simulink library "lib_LargeBuildingModel"  (R2026a)
settings: Solver=VariableStepAuto
libraries: WallSelector_lib x380, ExternalWall_lib x188, RoomWithAirVolume x140, fl_lib x139, RoomLevelControl_lib x1
(part 1 of 12)
settings Model: Creator=vikrants  LastModifiedBy=vikrants

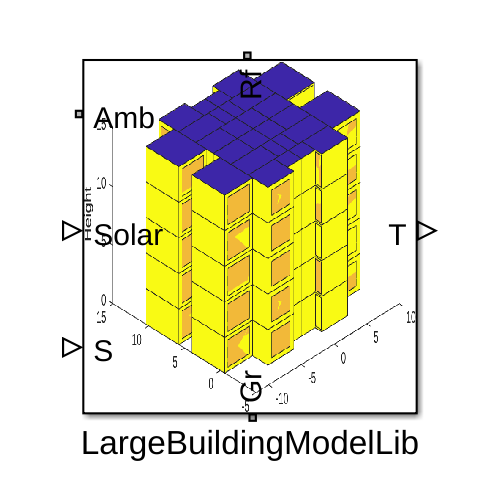
[thumbnail: Simulink's stored preview of the top-level diagram]
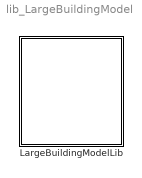
== system lib_LargeBuildingModel ==
  LargeBuildingModelLib : Subsystem
      settings: PortSchema="{\"entries\":[{\"content\":{\"sides\":[{\"content\":{\"connectorIds\":[\"LConn1\",\"LConn2\",\"LConn3\"]},\"type\":\"ConnectorPlacement.EquallySpacedRectSide\",\"uuid\":\"a54174e5-5a1e-4089-b263-99354bf7a073\"},{\"content\":{\"connectorIds\":[\"RConn1\"],\"side\":\"RIGHT\"},\"type\":\"ConnectorPlacement.EquallySpacedRectSide\",\"uuid\":\"c2c2a31f-cd98-4c14-b6c8-dd8555ba1cf6\"},{\"content\":{\"connectorIds\":[\"LConn4\"],\"side\":\"TOP\"},\"type\":\"ConnectorPlacement.EquallySpacedRectSide\",\"uuid\":\"2487b9c5-89a9-4b1a-9c1c-aa8a65c4be64\"},{\"content\":{\"connectorIds\":[\"RConn2\"],\"side\":\"BOTTOM\"},\"type\":\"ConnectorPlacement.EquallySpacedRectSide\",\"uuid\":\"6826558f-5b15-4554-8d35-ce4ee9628e1d\"}]},\"type\":\"ConnectorPlacement.EquallySpacedConnector\",\"uuid\":\"0b65bcf1-6575-4ff3-9247-4f08434b0bb6\"}],\"packageUris\":[\"http://schema.mathworks.com/mf0/Connector/R2020b\"],\"version\":\"1.0\"}"
      mask Display: image('lib_LargeBuildingModel.png')

== system lib_LargeBuildingModel/LargeBuildingModelLib ==
  ConnectLevel0and1 : Subsystem
      settings: PortSchema="{\"entries\":[{\"content\":{\"sides\":[{\"content\":{},\"type\":\"ConnectorPlacement.EquallySpacedRectSide\",\"uuid\":\"bfcbcdaf-7e68-43ba-b21b-739e3d917df2\"},{\"content\":{\"side\":\"RIGHT\"},\"type\":\"ConnectorPlacement.EquallySpacedRectSide\",\"uuid\":\"1db46710-465c-454f-9fe4-f8c04c90b155\"},{\"content\":{\"connectorIds\":[\"LConn1\"],\"side\":\"TOP\"},\"type\":\"ConnectorPlacement.EquallySpacedRectSide\",\"uuid\":\"8ba3322a-28ec-4bcd-a32b-78c0e69bc71f\"},{\"content\":{\"connectorIds\":[\"RConn1\"],\"side\":\"BOTTOM\"},\"type\":\"ConnectorPlacement.EquallySpacedRectSide\",\"uuid\":\"ab838286-00a0-4d85-b927-59d0a4342f32\"}]},\"type\":\"ConnectorPlacement.EquallySpacedConnector\",\"uuid\":\"bc7fd7cc-de66-4685-913a-91b57874b9ec\"}],\"packageUris\":[\"http://schema.mathworks.com/mf0/Connector/R2020b\"],\"version\":\"1.0\"}"
  ConnectLevel1and2 : Subsystem
      settings: PortSchema="{\"entries\":[{\"content\":{\"sides\":[{\"content\":{},\"type\":\"ConnectorPlacement.EquallySpacedRectSide\",\"uuid\":\"bfcbcdaf-7e68-43ba-b21b-739e3d917df2\"},{\"content\":{\"side\":\"RIGHT\"},\"type\":\"ConnectorPlacement.EquallySpacedRectSide\",\"uuid\":\"1db46710-465c-454f-9fe4-f8c04c90b155\"},{\"content\":{\"connectorIds\":[\"LConn1\"],\"side\":\"TOP\"},\"type\":\"ConnectorPlacement.EquallySpacedRectSide\",\"uuid\":\"8ba3322a-28ec-4bcd-a32b-78c0e69bc71f\"},{\"content\":{\"connectorIds\":[\"RConn1\"],\"side\":\"BOTTOM\"},\"type\":\"ConnectorPlacement.EquallySpacedRectSide\",\"uuid\":\"f3ab9cf8-9c6a-48e9-b20b-6fd302e3ecc9\"}]},\"type\":\"ConnectorPlacement.EquallySpacedConnector\",\"uuid\":\"bc7fd7cc-de66-4685-913a-91b57874b9ec\"}],\"packageUris\":[\"http://schema.mathworks.com/mf0/Connector/R2020b\"],\"version\":\"1.0\"}"
  ConnectLevel2and3 : Subsystem
      settings: PortSchema="{\"entries\":[{\"content\":{\"sides\":[{\"content\":{},\"type\":\"ConnectorPlacement.EquallySpacedRectSide\",\"uuid\":\"bfcbcdaf-7e68-43ba-b21b-739e3d917df2\"},{\"content\":{\"side\":\"RIGHT\"},\"type\":\"ConnectorPlacement.EquallySpacedRectSide\",\"uuid\":\"1db46710-465c-454f-9fe4-f8c04c90b155\"},{\"content\":{\"connectorIds\":[\"LConn1\"],\"side\":\"TOP\"},\"type\":\"ConnectorPlacement.EquallySpacedRectSide\",\"uuid\":\"8ba3322a-28ec-4bcd-a32b-78c0e69bc71f\"},{\"content\":{\"connectorIds\":[\"RConn1\"],\"side\":\"BOTTOM\"},\"type\":\"ConnectorPlacement.EquallySpacedRectSide\",\"uuid\":\"f8b3c343-7c17-4a2c-a5df-2d9e42135e3d\"}]},\"type\":\"ConnectorPlacement.EquallySpacedConnector\",\"uuid\":\"bc7fd7cc-de66-4685-913a-91b57874b9ec\"}],\"packageUris\":[\"http://schema.mathworks.com/mf0/Connector/R2020b\"],\"version\":\"1.0\"}"
  ConnectLevel3and4 : Subsystem
      settings: PortSchema="{\"entries\":[{\"content\":{\"sides\":[{\"content\":{},\"type\":\"ConnectorPlacement.EquallySpacedRectSide\",\"uuid\":\"bfcbcdaf-7e68-43ba-b21b-739e3d917df2\"},{\"content\":{\"side\":\"RIGHT\"},\"type\":\"ConnectorPlacement.EquallySpacedRectSide\",\"uuid\":\"1db46710-465c-454f-9fe4-f8c04c90b155\"},{\"content\":{\"connectorIds\":[\"LConn1\"],\"side\":\"TOP\"},\"type\":\"ConnectorPlacement.EquallySpacedRectSide\",\"uuid\":\"8ba3322a-28ec-4bcd-a32b-78c0e69bc71f\"},{\"content\":{\"connectorIds\":[\"RConn1\"],\"side\":\"BOTTOM\"},\"type\":\"ConnectorPlacement.EquallySpacedRectSide\",\"uuid\":\"2c50accd-6f19-4351-b387-00bd4c13865a\"}]},\"type\":\"ConnectorPlacement.EquallySpacedConnector\",\"uuid\":\"bc7fd7cc-de66-4685-913a-91b57874b9ec\"}],\"packageUris\":[\"http://schema.mathworks.com/mf0/Connector/R2020b\"],\"version\":\"1.0\"}"
  Ground : Subsystem
      settings: PortSchema="{\"entries\":[{\"content\":{\"sides\":[{\"content\":{},\"type\":\"ConnectorPlacement.EquallySpacedRectSide\",\"uuid\":\"bfcbcdaf-7e68-43ba-b21b-739e3d917df2\"},{\"content\":{\"side\":\"RIGHT\"},\"type\":\"ConnectorPlacement.EquallySpacedRectSide\",\"uuid\":\"1db46710-465c-454f-9fe4-f8c04c90b155\"},{\"content\":{\"connectorIds\":[\"LConn1\"],\"side\":\"TOP\"},\"type\":\"ConnectorPlacement.EquallySpacedRectSide\",\"uuid\":\"8ba3322a-28ec-4bcd-a32b-78c0e69bc71f\"},{\"content\":{\"connectorIds\":[\"RConn1\"],\"side\":\"BOTTOM\"},\"type\":\"ConnectorPlacement.EquallySpacedRectSide\",\"uuid\":\"e9de58ce-608e-4d22-b435-941c76f225f1\"}]},\"type\":\"ConnectorPlacement.EquallySpacedConnector\",\"uuid\":\"bc7fd7cc-de66-4685-913a-91b57874b9ec\"}],\"packageUris\":[\"http://schema.mathworks.com/mf0/Connector/R2020b\"],\"version\":\"1.0\"}"
  Level0 : Subsystem
      settings: PortSchema="{\"entries\":[{\"content\":{\"sides\":[{\"content\":{\"connectorIds\":[\"LConn1\",\"LConn2\",\"LConn3\"]},\"type\":\"ConnectorPlacement.EquallySpacedRectSide\",\"uuid\":\"f5302b38-994b-4d73-bed8-b19055c1e83a\"},{\"content\":{\"connectorIds\":[\"RConn1\"],\"side\":\"RIGHT\"},\"type\":\"ConnectorPlacement.EquallySpacedRectSide\",\"uuid\":\"faa5d083-f69a-475e-bab7-3d1e14a6968b\"},{\"content\":{\"connectorIds\":[\"LConn4\"],\"side\":\"TOP\"},\"type\":\"ConnectorPlacement.EquallySpacedRectSide\",\"uuid\":\"f79c44c3-41c3-478c-a059-469d9fb7ebbf\"},{\"content\":{\"connectorIds\":[\"RConn2\"],\"side\":\"BOTTOM\"},\"type\":\"ConnectorPlacement.EquallySpacedRectSide\",\"uuid\":\"9239f0d3-0017-4bc4-8897-67227729a1c7\"}]},\"type\":\"ConnectorPlacement.EquallySpacedConnector\",\"uuid\":\"c9eb4cc8-9d3a-4a18-b359-75861972c164\"}],\"packageUris\":[\"http://schema.mathworks.com/mf0/Connector/R2020b\"],\"version\":\"1.0\"}"
  Level1 : Subsystem
      settings: PortSchema="{\"entries\":[{\"content\":{\"sides\":[{\"content\":{\"connectorIds\":[\"LConn1\",\"LConn2\",\"LConn3\"]},\"type\":\"ConnectorPlacement.EquallySpacedRectSide\",\"uuid\":\"f5302b38-994b-4d73-bed8-b19055c1e83a\"},{\"content\":{\"connectorIds\":[\"RConn1\"],\"side\":\"RIGHT\"},\"type\":\"ConnectorPlacement.EquallySpacedRectSide\",\"uuid\":\"faa5d083-f69a-475e-bab7-3d1e14a6968b\"},{\"content\":{\"connectorIds\":[\"LConn4\"],\"side\":\"TOP\"},\"type\":\"ConnectorPlacement.EquallySpacedRectSide\",\"uuid\":\"f79c44c3-41c3-478c-a059-469d9fb7ebbf\"},{\"content\":{\"connectorIds\":[\"RConn2\"],\"side\":\"BOTTOM\"},\"type\":\"ConnectorPlacement.EquallySpacedRectSide\",\"uuid\":\"a0801537-0af0-4bd5-9c9a-f5991b45aca8\"}]},\"type\":\"ConnectorPlacement.EquallySpacedConnector\",\"uuid\":\"c9eb4cc8-9d3a-4a18-b359-75861972c164\"}],\"packageUris\":[\"http://schema.mathworks.com/mf0/Connector/R2020b\"],\"version\":\"1.0\"}"
  Level2 : Subsystem
      settings: PortSchema="{\"entries\":[{\"content\":{\"sides\":[{\"content\":{\"connectorIds\":[\"LConn1\",\"LConn2\",\"LConn3\"]},\"type\":\"ConnectorPlacement.EquallySpacedRectSide\",\"uuid\":\"f5302b38-994b-4d73-bed8-b19055c1e83a\"},{\"content\":{\"connectorIds\":[\"RConn1\"],\"side\":\"RIGHT\"},\"type\":\"ConnectorPlacement.EquallySpacedRectSide\",\"uuid\":\"faa5d083-f69a-475e-bab7-3d1e14a6968b\"},{\"content\":{\"connectorIds\":[\"LConn4\"],\"side\":\"TOP\"},\"type\":\"ConnectorPlacement.EquallySpacedRectSide\",\"uuid\":\"f79c44c3-41c3-478c-a059-469d9fb7ebbf\"},{\"content\":{\"connectorIds\":[\"RConn2\"],\"side\":\"BOTTOM\"},\"type\":\"ConnectorPlacement.EquallySpacedRectSide\",\"uuid\":\"bd08f839-c923-45c8-997c-e7bb9423b19d\"}]},\"type\":\"ConnectorPlacement.EquallySpacedConnector\",\"uuid\":\"c9eb4cc8-9d3a-4a18-b359-75861972c164\"}],\"packageUris\":[\"http://schema.mathworks.com/mf0/Connector/R2020b\"],\"version\":\"1.0\"}"
  Level3 : Subsystem
      settings: PortSchema="{\"entries\":[{\"content\":{\"sides\":[{\"content\":{\"connectorIds\":[\"LConn1\",\"LConn2\",\"LConn3\"]},\"type\":\"ConnectorPlacement.EquallySpacedRectSide\",\"uuid\":\"f5302b38-994b-4d73-bed8-b19055c1e83a\"},{\"content\":{\"connectorIds\":[\"RConn1\"],\"side\":\"RIGHT\"},\"type\":\"ConnectorPlacement.EquallySpacedRectSide\",\"uuid\":\"faa5d083-f69a-475e-bab7-3d1e14a6968b\"},{\"content\":{\"connectorIds\":[\"LConn4\"],\"side\":\"TOP\"},\"type\":\"ConnectorPlacement.EquallySpacedRectSide\",\"uuid\":\"f79c44c3-41c3-478c-a059-469d9fb7ebbf\"},{\"content\":{\"connectorIds\":[\"RConn2\"],\"side\":\"BOTTOM\"},\"type\":\"ConnectorPlacement.EquallySpacedRectSide\",\"uuid\":\"6ad92d71-3c8c-43ae-8be8-bbeacb5a4479\"}]},\"type\":\"ConnectorPlacement.EquallySpacedConnector\",\"uuid\":\"c9eb4cc8-9d3a-4a18-b359-75861972c164\"}],\"packageUris\":[\"http://schema.mathworks.com/mf0/Connector/R2020b\"],\"version\":\"1.0\"}"
  Level4 : Subsystem
      settings: PortSchema="{\"entries\":[{\"content\":{\"sides\":[{\"content\":{\"connectorIds\":[\"LConn1\",\"LConn2\",\"LConn3\"]},\"type\":\"ConnectorPlacement.EquallySpacedRectSide\",\"uuid\":\"f5302b38-994b-4d73-bed8-b19055c1e83a\"},{\"content\":{\"connectorIds\":[\"RConn1\"],\"side\":\"RIGHT\"},\"type\":\"ConnectorPlacement.EquallySpacedRectSide\",\"uuid\":\"faa5d083-f69a-475e-bab7-3d1e14a6968b\"},{\"content\":{\"connectorIds\":[\"LConn4\"],\"side\":\"TOP\"},\"type\":\"ConnectorPlacement.EquallySpacedRectSide\",\"uuid\":\"f79c44c3-41c3-478c-a059-469d9fb7ebbf\"},{\"content\":{\"connectorIds\":[\"RConn2\"],\"side\":\"BOTTOM\"},\"type\":\"ConnectorPlacement.EquallySpacedRectSide\",\"uuid\":\"444ccc88-7c7b-4932-a02b-9df645918112\"}]},\"type\":\"ConnectorPlacement.EquallySpacedConnector\",\"uuid\":\"c9eb4cc8-9d3a-4a18-b359-75861972c164\"}],\"packageUris\":[\"http://schema.mathworks.com/mf0/Connector/R2020b\"],\"version\":\"1.0\"}"
  Roof : Subsystem
      settings: PortSchema="{\"entries\":[{\"content\":{\"sides\":[{\"content\":{\"connectorIds\":[\"LConn1\"]},\"type\":\"ConnectorPlacement.EquallySpacedRectSide\",\"uuid\":\"330a1f4c-788b-45d3-8144-461e13e4bc2b\"},{\"content\":{\"side\":\"RIGHT\"},\"type\":\"ConnectorPlacement.EquallySpacedRectSide\",\"uuid\":\"2ff68f0e-d161-486d-a47e-10633b293a9f\"},{\"content\":{\"connectorIds\":[\"LConn2\"],\"side\":\"TOP\"},\"type\":\"ConnectorPlacement.EquallySpacedRectSide\",\"uuid\":\"a18254b5-007e-4575-8004-ea2058ac2122\"},{\"content\":{\"connectorIds\":[\"RConn1\"],\"side\":\"BOTTOM\"},\"type\":\"ConnectorPlacement.EquallySpacedRectSide\",\"uuid\":\"9d9d06c4-f9b4-44db-a6ff-ed6ffbc85269\"}]},\"type\":\"ConnectorPlacement.EquallySpacedConnector\",\"uuid\":\"c0f19b20-ad71-4ed9-8cf3-6c486454730f\"}],\"packageUris\":[\"http://schema.mathworks.com/mf0/Connector/R2020b\"],\"version\":\"1.0\"}"
  Sv : RoomLevelControl_lib/Room Level Control  portOption=roomControlOption.heat  roomMapping=[1 1 1 1;1 1 2 2;1 1 3 3;1 1 4 4;1 1 5 5;1 1 6 6;1 1 7 7;1 2 1 8;1 2 2 9;1 2 3 10;1 2 4 11;1 2 5 12;1 2 6 13;1 2 7 14;1 3 1 15;1 3 2 16;1 3 3 17;1 3 4 18;1 3 5 19;1 3 6 20;1 3 7 21;1 4 1 22;1 4 2 23;1 4 3 24;1 4 4 25;1 4 5 26;1 4 6 27;1 4 7 28;2 5 1 29;2 5 2 30;2 5 3 31;2 5 4 32;2 5 5 33;2 5 6 34;2 5 7 35;2 6 1 36;2 6 2 37;2 6 3 38;2 6 4 39;2 6 5 40;2 6 6 41;2 6 7 42;2 7 1 43;2 7 2 44;2 7 3 45;2 7 4 46;2 7 5 47;2 7 6 48;2 7 7 49;2 8 1 50;2 8 2 51;2 8 3 52;2 8 4 53;2 8 5 54;2 8 6 55;2 8 7 56;3 9 1 57;3 9 2 58;3 9 3 59;3 9 4 60;3 9 5 61;3 9 6 62;3 9 7 63;3 10 1 64;3 10 2 65;3 10 3 66;3 10 4 67;3 10 5 68;3 10 6 69;3 10 7 70;3 11 1 71;3 11 2 72;3 11 3 73;3 11 4 74;3 11 5 75;3 11 6 76;3 11 7 77;3 12 1 78;3 12 2 79;3 12 3 80;3 12 4 81;3 12 5 82;3 12 6 83;3 12 7 84;4 13 1 85;4 13 2 86;4 13 3 87;4 13 4 88;4 13 5 89;4 13 6 90;4 13 7 91;4 14 1 92;4 14 2 93;4 14 3 94;4 14 4 95;4 14 5 96;4 14 6 97;4 14 7 98;4 15 1 99;4 15 2 100;4 15 3 101;4 15 4 102;4 15 5 103;4 15 6 104;4 15 7 105;4 16 1 106;4 16 2 107;4 16 3 108;4 16 4 109;4 16 5 110;4 16 6 111;4 16 7 112;5 17 1 113;5 17 2 114;5 17 3 115;5 17 4 116;5 17 5 117;5 17 6 118;5 17 7 119;5 18 1 120;5 18 2 121;5 18 3 122;5 18 4 123;5 18 5 124;5 18 6 125;5 18 7 126;5 19 1 127;5 19 2 128;5 19 3 129;5 19 4 130;5 19 5 131;5 19 6 132;5 19 7 133;5 20 1 134;5 20 2 135;5 20 3 136;5 20 4 137;5 20 5 138;5 20 6 139;5 20 7 140]
  roomT : Subsystem
  Amb : PMIOPort  Side=Left
  Solar : PMIOPort  Port=2  Side=Left
  S : PMIOPort  Port=3  Side=Left
  Rf : PMIOPort  Port=4  Side=Left
  T : PMIOPort  Port=5  Side=Right
  Gr : PMIOPort  Port=6  Side=Right
  connections:
  Level0/RConn2 -- Ground/LConn1
  Level1/RConn2 -- ConnectLevel0and1/LConn1
  Level0/LConn4 -- ConnectLevel0and1/RConn1
  Level2/RConn2 -- ConnectLevel1and2/LConn1
  Level1/LConn4 -- ConnectLevel1and2/RConn1
  Level3/RConn2 -- ConnectLevel2and3/LConn1
  Level2/LConn4 -- ConnectLevel2and3/RConn1
  Level4/RConn2 -- ConnectLevel3and4/LConn1
  Level3/LConn4 -- ConnectLevel3and4/RConn1
  Level4/LConn4 -- Roof/RConn1
  Sv/LConn1 -- S/RConn1
  Roof/LConn2 -- Rf/RConn1
  Ground/RConn1 -- Gr/RConn1
  Roof/LConn1 -- Level0/LConn2 -- Level1/LConn2 -- Level2/LConn2 -- Level3/LConn2 -- Solar/RConn1 -- Level4/LConn2
  Level0/LConn1 -- Level1/LConn1 -- Level2/LConn1 -- Level3/LConn1 -- Amb/RConn1 -- Level4/LConn1
  Level0/LConn3 -- Level1/LConn3 -- Level2/LConn3 -- Level3/LConn3 -- Sv/RConn1 -- Level4/LConn3
  roomT/LConn1 -- Level0/RConn1
  roomT/LConn2 -- Level1/RConn1
  roomT/LConn3 -- Level2/RConn1
  roomT/LConn4 -- Level3/RConn1
  roomT/LConn5 -- Level4/RConn1
  roomT/RConn1 -- T/RConn1

== system lib_LargeBuildingModel/LargeBuildingModelLib/ConnectLevel0and1 ==
  note: Floor_A1R1(LivingRoom_A)
  note: Floor_A1R2(Bedroom_A)
  note: Floor_A1R3(Kitchen_A)
  note: Floor_A1R4(Bathroom_A)
  note: Floor_A1R5(FireExit_A)
  note: Floor_A1R6(Lobby1_A)
  note: Floor_A1R7(Lobby2_A)
  note: Floor_A2R1(LivingRoom_B)
  note: Floor_A2R2(Bedroom_B)
  note: Floor_A2R3(Kitchen_B)
  note: Floor_A2R4(Bathroom_B)
  note: Floor_A2R5(FireExit_B)
  note: Floor_A2R6(Lobby1_B)
  note: Floor_A2R7(Lobby2_B)
  note: Floor_A3R1(LivingRoom_C)
  note: Floor_A3R2(Bedroom_C)
  note: Floor_A3R3(Kitchen_C)
  note: Floor_A3R4(Bathroom_C)
  note: Floor_A3R5(FireExit_C)
  note: Floor_A3R6(Lobby1_C)
  note: Floor_A3R7(Lobby2_C)
  note: Floor_A4R1(LivingRoom_D)
  note: Floor_A4R2(Bedroom_D)
  note: Floor_A4R3(Kitchen_D)
  note: Floor_A4R4(Bathroom_D)
  note: Floor_A4R5(FireExit_D)
  note: Floor_A4R6(Lobby1_D)
  note: Floor_A4R7(Lobby2_D)
  ArrayBottom : SimscapeArrayConnection  Domain=foundation.thermal.thermal  ConcatenateDimension=1  NumScalarElements=28
  ArrayTop : SimscapeArrayConnection  Domain=foundation.thermal.thermal  ConcatenateDimension=1  NumScalarElements=28
  Floor_A1R1(LivingRoom_A)Blk : WallSelector_lib/Wall Selector  optWall=wallModelOption.wallOnly  wallLength=2.4384 % Parameterized on : 13-Jun-2026 10:47:15 m  wallHeight=4.572 % Parameterized on : 13-Jun-2026 10:47:15 m  wallThickness=0.03 % Parameterized on : 13-Jun-2026 10:47:15 m  wallMaterialDen=1400 % Parameterized on : 13-Jun-2026 10:47:28 kg/m^3  wallMaterialCp=1000 % Parameterized on : 13-Jun-2026 10:47:28 J/(K*kg)  wallAbsorptivity=0.5  wallThermalK=0.7 % Parameterized on : 13-Jun-2026 10:47:28 W/(K*m)  winLength=1 m  winHeight=0.5 m  winThickness=0.007 m  winMaterialDen=2500 kg/m^3  winMaterialCp=787 J/(K*kg)  winAbsorptivity=0.35  winThermalK=1 W/(K*m)  winTransmissivity=0.45  ventLength=0.1 m  ventHeight=0.1 m  extToWallHTC=30 % Parameterized on : 13-Jun-2026 10:47:28 W/(K*m^2)  intToRoomHTC=30 % Parameterized on : 13-Jun-2026 10:47:28 W/(K*m^2)  iniT=300 % Parameterized on : 13-Jun-2026 10:47:28 K
  Floor_A1R2(Bedroom_A)Blk : WallSelector_lib/Wall Selector  optWall=wallModelOption.wallOnly  wallLength=4.2672 % Parameterized on : 13-Jun-2026 10:47:15 m  wallHeight=4.572 % Parameterized on : 13-Jun-2026 10:47:15 m  wallThickness=0.03 % Parameterized on : 13-Jun-2026 10:47:15 m  wallMaterialDen=1400 % Parameterized on : 13-Jun-2026 10:47:28 kg/m^3  wallMaterialCp=1000 % Parameterized on : 13-Jun-2026 10:47:28 J/(K*kg)  wallAbsorptivity=0.5  wallThermalK=0.7 % Parameterized on : 13-Jun-2026 10:47:28 W/(K*m)  winLength=1 m  winHeight=0.5 m  winThickness=0.007 m  winMaterialDen=2500 kg/m^3  winMaterialCp=787 J/(K*kg)  winAbsorptivity=0.35  winThermalK=1 W/(K*m)  winTransmissivity=0.45  ventLength=0.1 m  ventHeight=0.1 m  extToWallHTC=30 % Parameterized on : 13-Jun-2026 10:47:28 W/(K*m^2)  intToRoomHTC=30 % Parameterized on : 13-Jun-2026 10:47:28 W/(K*m^2)  iniT=300 % Parameterized on : 13-Jun-2026 10:47:28 K
  Floor_A1R3(Kitchen_A)Blk : WallSelector_lib/Wall Selector  optWall=wallModelOption.wallOnly  wallLength=2.7432 % Parameterized on : 13-Jun-2026 10:47:15 m  wallHeight=3.9624 % Parameterized on : 13-Jun-2026 10:47:15 m  wallThickness=0.03 % Parameterized on : 13-Jun-2026 10:47:15 m  wallMaterialDen=1400 % Parameterized on : 13-Jun-2026 10:47:28 kg/m^3  wallMaterialCp=1000 % Parameterized on : 13-Jun-2026 10:47:28 J/(K*kg)  wallAbsorptivity=0.5  wallThermalK=0.7 % Parameterized on : 13-Jun-2026 10:47:28 W/(K*m)  winLength=1 m  winHeight=0.5 m  winThickness=0.007 m  winMaterialDen=2500 kg/m^3  winMaterialCp=787 J/(K*kg)  winAbsorptivity=0.35  winThermalK=1 W/(K*m)  winTransmissivity=0.45  ventLength=0.1 m  ventHeight=0.1 m  extToWallHTC=30 % Parameterized on : 13-Jun-2026 10:47:28 W/(K*m^2)  intToRoomHTC=30 % Parameterized on : 13-Jun-2026 10:47:28 W/(K*m^2)  iniT=300 % Parameterized on : 13-Jun-2026 10:47:28 K
  Floor_A1R4(Bathroom_A)Blk : WallSelector_lib/Wall Selector  optWall=wallModelOption.wallOnly  wallLength=2.4384 % Parameterized on : 13-Jun-2026 10:47:15 m  wallHeight=3.6576 % Parameterized on : 13-Jun-2026 10:47:15 m  wallThickness=0.03 % Parameterized on : 13-Jun-2026 10:47:15 m  wallMaterialDen=1400 % Parameterized on : 13-Jun-2026 10:47:28 kg/m^3  wallMaterialCp=1000 % Parameterized on : 13-Jun-2026 10:47:28 J/(K*kg)  wallAbsorptivity=0.5  wallThermalK=0.7 % Parameterized on : 13-Jun-2026 10:47:28 W/(K*m)  winLength=1 m  winHeight=0.5 m  winThickness=0.007 m  winMaterialDen=2500 kg/m^3  winMaterialCp=787 J/(K*kg)  winAbsorptivity=0.35  winThermalK=1 W/(K*m)  winTransmissivity=0.45  ventLength=0.1 m  ventHeight=0.1 m  extToWallHTC=30 % Parameterized on : 13-Jun-2026 10:47:28 W/(K*m^2)  intToRoomHTC=30 % Parameterized on : 13-Jun-2026 10:47:28 W/(K*m^2)  iniT=300 % Parameterized on : 13-Jun-2026 10:47:28 K
  Floor_A1R5(FireExit_A)Blk : WallSelector_lib/Wall Selector  optWall=wallModelOption.wallOnly  wallLength=1.8288 % Parameterized on : 13-Jun-2026 10:47:15 m  wallHeight=2.1336 % Parameterized on : 13-Jun-2026 10:47:15 m  wallThickness=0.03 % Parameterized on : 13-Jun-2026 10:47:15 m  wallMaterialDen=1400 % Parameterized on : 13-Jun-2026 10:47:28 kg/m^3  wallMaterialCp=1000 % Parameterized on : 13-Jun-2026 10:47:28 J/(K*kg)  wallAbsorptivity=0.5  wallThermalK=0.7 % Parameterized on : 13-Jun-2026 10:47:28 W/(K*m)  winLength=1 m  winHeight=0.5 m  winThickness=0.007 m  winMaterialDen=2500 kg/m^3  winMaterialCp=787 J/(K*kg)  winAbsorptivity=0.35  winThermalK=1 W/(K*m)  winTransmissivity=0.45  ventLength=0.1 m  ventHeight=0.1 m  extToWallHTC=30 % Parameterized on : 13-Jun-2026 10:47:28 W/(K*m^2)  intToRoomHTC=30 % Parameterized on : 13-Jun-2026 10:47:28 W/(K*m^2)  iniT=300 % Parameterized on : 13-Jun-2026 10:47:28 K
  Floor_A1R6(Lobby1_A)Blk : WallSelector_lib/Wall Selector  optWall=wallModelOption.wallOnly  wallLength=2.4384 % Parameterized on : 13-Jun-2026 10:47:15 m  wallHeight=2.4384 % Parameterized on : 13-Jun-2026 10:47:15 m  wallThickness=0.03 % Parameterized on : 13-Jun-2026 10:47:15 m  wallMaterialDen=1400 % Parameterized on : 13-Jun-2026 10:47:28 kg/m^3  wallMaterialCp=1000 % Parameterized on : 13-Jun-2026 10:47:28 J/(K*kg)  wallAbsorptivity=0.5  wallThermalK=0.7 % Parameterized on : 13-Jun-2026 10:47:28 W/(K*m)  winLength=1 m  winHeight=0.5 m  winThickness=0.007 m  winMaterialDen=2500 kg/m^3  winMaterialCp=787 J/(K*kg)  winAbsorptivity=0.35  winThermalK=1 W/(K*m)  winTransmissivity=0.45  ventLength=0.1 m  ventHeight=0.1 m  extToWallHTC=30 % Parameterized on : 13-Jun-2026 10:47:28 W/(K*m^2)  intToRoomHTC=30 % Parameterized on : 13-Jun-2026 10:47:28 W/(K*m^2)  iniT=300 % Parameterized on : 13-Jun-2026 10:47:28 K
  Floor_A1R7(Lobby2_A)Blk : WallSelector_lib/Wall Selector  optWall=wallModelOption.wallOnly  wallLength=2.4384 % Parameterized on : 13-Jun-2026 10:47:15 m  wallHeight=1.524 % Parameterized on : 13-Jun-2026 10:47:15 m  wallThickness=0.03 % Parameterized on : 13-Jun-2026 10:47:15 m  wallMaterialDen=1400 % Parameterized on : 13-Jun-2026 10:47:28 kg/m^3  wallMaterialCp=1000 % Parameterized on : 13-Jun-2026 10:47:28 J/(K*kg)  wallAbsorptivity=0.5  wallThermalK=0.7 % Parameterized on : 13-Jun-2026 10:47:28 W/(K*m)  winLength=1 m  winHeight=0.5 m  winThickness=0.007 m  winMaterialDen=2500 kg/m^3  winMaterialCp=787 J/(K*kg)  winAbsorptivity=0.35  winThermalK=1 W/(K*m)  winTransmissivity=0.45  ventLength=0.1 m  ventHeight=0.1 m  extToWallHTC=30 % Parameterized on : 13-Jun-2026 10:47:28 W/(K*m^2)  intToRoomHTC=30 % Parameterized on : 13-Jun-2026 10:47:28 W/(K*m^2)  iniT=300 % Parameterized on : 13-Jun-2026 10:47:28 K
  Floor_A2R1(LivingRoom_B)Blk : WallSelector_lib/Wall Selector  optWall=wallModelOption.wallOnly  wallLength=2.4384 % Parameterized on : 13-Jun-2026 10:47:15 m  wallHeight=4.572 % Parameterized on : 13-Jun-2026 10:47:15 m  wallThickness=0.03 % Parameterized on : 13-Jun-2026 10:47:15 m  wallMaterialDen=1400 % Parameterized on : 13-Jun-2026 10:47:29 kg/m^3  wallMaterialCp=1000 % Parameterized on : 13-Jun-2026 10:47:29 J/(K*kg)  wallAbsorptivity=0.5  wallThermalK=0.7 % Parameterized on : 13-Jun-2026 10:47:29 W/(K*m)  winLength=1 m  winHeight=0.5 m  winThickness=0.007 m  winMaterialDen=2500 kg/m^3  winMaterialCp=787 J/(K*kg)  winAbsorptivity=0.35  winThermalK=1 W/(K*m)  winTransmissivity=0.45  ventLength=0.1 m  ventHeight=0.1 m  extToWallHTC=30 % Parameterized on : 13-Jun-2026 10:47:29 W/(K*m^2)  intToRoomHTC=30 % Parameterized on : 13-Jun-2026 10:47:29 W/(K*m^2)  iniT=300 % Parameterized on : 13-Jun-2026 10:47:29 K
  Floor_A2R2(Bedroom_B)Blk : WallSelector_lib/Wall Selector  optWall=wallModelOption.wallOnly  wallLength=4.2672 % Parameterized on : 13-Jun-2026 10:47:15 m  wallHeight=4.572 % Parameterized on : 13-Jun-2026 10:47:15 m  wallThickness=0.03 % Parameterized on : 13-Jun-2026 10:47:15 m  wallMaterialDen=1400 % Parameterized on : 13-Jun-2026 10:47:29 kg/m^3  wallMaterialCp=1000 % Parameterized on : 13-Jun-2026 10:47:29 J/(K*kg)  wallAbsorptivity=0.5  wallThermalK=0.7 % Parameterized on : 13-Jun-2026 10:47:29 W/(K*m)  winLength=1 m  winHeight=0.5 m  winThickness=0.007 m  winMaterialDen=2500 kg/m^3  winMaterialCp=787 J/(K*kg)  winAbsorptivity=0.35  winThermalK=1 W/(K*m)  winTransmissivity=0.45  ventLength=0.1 m  ventHeight=0.1 m  extToWallHTC=30 % Parameterized on : 13-Jun-2026 10:47:29 W/(K*m^2)  intToRoomHTC=30 % Parameterized on : 13-Jun-2026 10:47:29 W/(K*m^2)  iniT=300 % Parameterized on : 13-Jun-2026 10:47:29 K
  Floor_A2R3(Kitchen_B)Blk : WallSelector_lib/Wall Selector  optWall=wallModelOption.wallOnly  wallLength=2.7432 % Parameterized on : 13-Jun-2026 10:47:15 m  wallHeight=3.9624 % Parameterized on : 13-Jun-2026 10:47:15 m  wallThickness=0.03 % Parameterized on : 13-Jun-2026 10:47:15 m  wallMaterialDen=1400 % Parameterized on : 13-Jun-2026 10:47:29 kg/m^3  wallMaterialCp=1000 % Parameterized on : 13-Jun-2026 10:47:29 J/(K*kg)  wallAbsorptivity=0.5  wallThermalK=0.7 % Parameterized on : 13-Jun-2026 10:47:29 W/(K*m)  winLength=1 m  winHeight=0.5 m  winThickness=0.007 m  winMaterialDen=2500 kg/m^3  winMaterialCp=787 J/(K*kg)  winAbsorptivity=0.35  winThermalK=1 W/(K*m)  winTransmissivity=0.45  ventLength=0.1 m  ventHeight=0.1 m  extToWallHTC=30 % Parameterized on : 13-Jun-2026 10:47:29 W/(K*m^2)  intToRoomHTC=30 % Parameterized on : 13-Jun-2026 10:47:29 W/(K*m^2)  iniT=300 % Parameterized on : 13-Jun-2026 10:47:29 K
  Floor_A2R4(Bathroom_B)Blk : WallSelector_lib/Wall Selector  optWall=wallModelOption.wallOnly  wallLength=2.4384 % Parameterized on : 13-Jun-2026 10:47:15 m  wallHeight=3.6576 % Parameterized on : 13-Jun-2026 10:47:15 m  wallThickness=0.03 % Parameterized on : 13-Jun-2026 10:47:15 m  wallMaterialDen=1400 % Parameterized on : 13-Jun-2026 10:47:29 kg/m^3  wallMaterialCp=1000 % Parameterized on : 13-Jun-2026 10:47:29 J/(K*kg)  wallAbsorptivity=0.5  wallThermalK=0.7 % Parameterized on : 13-Jun-2026 10:47:29 W/(K*m)  winLength=1 m  winHeight=0.5 m  winThickness=0.007 m  winMaterialDen=2500 kg/m^3  winMaterialCp=787 J/(K*kg)  winAbsorptivity=0.35  winThermalK=1 W/(K*m)  winTransmissivity=0.45  ventLength=0.1 m  ventHeight=0.1 m  extToWallHTC=30 % Parameterized on : 13-Jun-2026 10:47:29 W/(K*m^2)  intToRoomHTC=30 % Parameterized on : 13-Jun-2026 10:47:29 W/(K*m^2)  iniT=300 % Parameterized on : 13-Jun-2026 10:47:29 K
  Floor_A2R5(FireExit_B)Blk : WallSelector_lib/Wall Selector  optWall=wallModelOption.wallOnly  wallLength=1.8288 % Parameterized on : 13-Jun-2026 10:47:15 m  wallHeight=2.1336 % Parameterized on : 13-Jun-2026 10:47:15 m  wallThickness=0.03 % Parameterized on : 13-Jun-2026 10:47:15 m  wallMaterialDen=1400 % Parameterized on : 13-Jun-2026 10:47:29 kg/m^3  wallMaterialCp=1000 % Parameterized on : 13-Jun-2026 10:47:29 J/(K*kg)  wallAbsorptivity=0.5  wallThermalK=0.7 % Parameterized on : 13-Jun-2026 10:47:29 W/(K*m)  winLength=1 m  winHeight=0.5 m  winThickness=0.007 m  winMaterialDen=2500 kg/m^3  winMaterialCp=787 J/(K*kg)  winAbsorptivity=0.35  winThermalK=1 W/(K*m)  winTransmissivity=0.45  ventLength=0.1 m  ventHeight=0.1 m  extToWallHTC=30 % Parameterized on : 13-Jun-2026 10:47:29 W/(K*m^2)  intToRoomHTC=30 % Parameterized on : 13-Jun-2026 10:47:29 W/(K*m^2)  iniT=300 % Parameterized on : 13-Jun-2026 10:47:29 K
  Floor_A2R6(Lobby1_B)Blk : WallSelector_lib/Wall Selector  optWall=wallModelOption.wallOnly  wallLength=2.4384 % Parameterized on : 13-Jun-2026 10:47:15 m  wallHeight=2.4384 % Parameterized on : 13-Jun-2026 10:47:15 m  wallThickness=0.03 % Parameterized on : 13-Jun-2026 10:47:15 m  wallMaterialDen=1400 % Parameterized on : 13-Jun-2026 10:47:29 kg/m^3  wallMaterialCp=1000 % Parameterized on : 13-Jun-2026 10:47:29 J/(K*kg)  wallAbsorptivity=0.5  wallThermalK=0.7 % Parameterized on : 13-Jun-2026 10:47:29 W/(K*m)  winLength=1 m  winHeight=0.5 m  winThickness=0.007 m  winMaterialDen=2500 kg/m^3  winMaterialCp=787 J/(K*kg)  winAbsorptivity=0.35  winThermalK=1 W/(K*m)  winTransmissivity=0.45  ventLength=0.1 m  ventHeight=0.1 m  extToWallHTC=30 % Parameterized on : 13-Jun-2026 10:47:29 W/(K*m^2)  intToRoomHTC=30 % Parameterized on : 13-Jun-2026 10:47:29 W/(K*m^2)  iniT=300 % Parameterized on : 13-Jun-2026 10:47:29 K
  Floor_A2R7(Lobby2_B)Blk : WallSelector_lib/Wall Selector  optWall=wallModelOption.wallOnly  wallLength=2.4384 % Parameterized on : 13-Jun-2026 10:47:15 m  wallHeight=1.524 % Parameterized on : 13-Jun-2026 10:47:15 m  wallThickness=0.03 % Parameterized on : 13-Jun-2026 10:47:15 m  wallMaterialDen=1400 % Parameterized on : 13-Jun-2026 10:47:29 kg/m^3  wallMaterialCp=1000 % Parameterized on : 13-Jun-2026 10:47:29 J/(K*kg)  wallAbsorptivity=0.5  wallThermalK=0.7 % Parameterized on : 13-Jun-2026 10:47:29 W/(K*m)  winLength=1 m  winHeight=0.5 m  winThickness=0.007 m  winMaterialDen=2500 kg/m^3  winMaterialCp=787 J/(K*kg)  winAbsorptivity=0.35  winThermalK=1 W/(K*m)  winTransmissivity=0.45  ventLength=0.1 m  ventHeight=0.1 m  extToWallHTC=30 % Parameterized on : 13-Jun-2026 10:47:29 W/(K*m^2)  intToRoomHTC=30 % Parameterized on : 13-Jun-2026 10:47:29 W/(K*m^2)  iniT=300 % Parameterized on : 13-Jun-2026 10:47:29 K
  Floor_A3R1(LivingRoom_C)Blk : WallSelector_lib/Wall Selector  optWall=wallModelOption.wallOnly  wallLength=2.4384 % Parameterized on : 13-Jun-2026 10:47:15 m  wallHeight=4.572 % Parameterized on : 13-Jun-2026 10:47:15 m  wallThickness=0.03 % Parameterized on : 13-Jun-2026 10:47:15 m  wallMaterialDen=1400 % Parameterized on : 13-Jun-2026 10:47:29 kg/m^3  wallMaterialCp=1000 % Parameterized on : 13-Jun-2026 10:47:29 J/(K*kg)  wallAbsorptivity=0.5  wallThermalK=0.7 % Parameterized on : 13-Jun-2026 10:47:29 W/(K*m)  winLength=1 m  winHeight=0.5 m  winThickness=0.007 m  winMaterialDen=2500 kg/m^3  winMaterialCp=787 J/(K*kg)  winAbsorptivity=0.35  winThermalK=1 W/(K*m)  winTransmissivity=0.45  ventLength=0.1 m  ventHeight=0.1 m  extToWallHTC=30 % Parameterized on : 13-Jun-2026 10:47:29 W/(K*m^2)  intToRoomHTC=30 % Parameterized on : 13-Jun-2026 10:47:29 W/(K*m^2)  iniT=300 % Parameterized on : 13-Jun-2026 10:47:29 K
  Floor_A3R2(Bedroom_C)Blk : WallSelector_lib/Wall Selector  optWall=wallModelOption.wallOnly  wallLength=4.2672 % Parameterized on : 13-Jun-2026 10:47:15 m  wallHeight=4.572 % Parameterized on : 13-Jun-2026 10:47:15 m  wallThickness=0.03 % Parameterized on : 13-Jun-2026 10:47:15 m  wallMaterialDen=1400 % Parameterized on : 13-Jun-2026 10:47:29 kg/m^3  wallMaterialCp=1000 % Parameterized on : 13-Jun-2026 10:47:29 J/(K*kg)  wallAbsorptivity=0.5  wallThermalK=0.7 % Parameterized on : 13-Jun-2026 10:47:29 W/(K*m)  winLength=1 m  winHeight=0.5 m  winThickness=0.007 m  winMaterialDen=2500 kg/m^3  winMaterialCp=787 J/(K*kg)  winAbsorptivity=0.35  winThermalK=1 W/(K*m)  winTransmissivity=0.45  ventLength=0.1 m  ventHeight=0.1 m  extToWallHTC=30 % Parameterized on : 13-Jun-2026 10:47:29 W/(K*m^2)  intToRoomHTC=30 % Parameterized on : 13-Jun-2026 10:47:29 W/(K*m^2)  iniT=300 % Parameterized on : 13-Jun-2026 10:47:29 K
  Floor_A3R3(Kitchen_C)Blk : WallSelector_lib/Wall Selector  optWall=wallModelOption.wallOnly  wallLength=2.7432 % Parameterized on : 13-Jun-2026 10:47:15 m  wallHeight=3.9624 % Parameterized on : 13-Jun-2026 10:47:15 m  wallThickness=0.03 % Parameterized on : 13-Jun-2026 10:47:15 m  wallMaterialDen=1400 % Parameterized on : 13-Jun-2026 10:47:29 kg/m^3  wallMaterialCp=1000 % Parameterized on : 13-Jun-2026 10:47:29 J/(K*kg)  wallAbsorptivity=0.5  wallThermalK=0.7 % Parameterized on : 13-Jun-2026 10:47:29 W/(K*m)  winLength=1 m  winHeight=0.5 m  winThickness=0.007 m  winMaterialDen=2500 kg/m^3  winMaterialCp=787 J/(K*kg)  winAbsorptivity=0.35  winThermalK=1 W/(K*m)  winTransmissivity=0.45  ventLength=0.1 m  ventHeight=0.1 m  extToWallHTC=30 % Parameterized on : 13-Jun-2026 10:47:29 W/(K*m^2)  intToRoomHTC=30 % Parameterized on : 13-Jun-2026 10:47:29 W/(K*m^2)  iniT=300 % Parameterized on : 13-Jun-2026 10:47:29 K
  Floor_A3R4(Bathroom_C)Blk : WallSelector_lib/Wall Selector  optWall=wallModelOption.wallOnly  wallLength=2.4384 % Parameterized on : 13-Jun-2026 10:47:15 m  wallHeight=3.6576 % Parameterized on : 13-Jun-2026 10:47:15 m  wallThickness=0.03 % Parameterized on : 13-Jun-2026 10:47:15 m  wallMaterialDen=1400 % Parameterized on : 13-Jun-2026 10:47:29 kg/m^3  wallMaterialCp=1000 % Parameterized on : 13-Jun-2026 10:47:29 J/(K*kg)  wallAbsorptivity=0.5  wallThermalK=0.7 % Parameterized on : 13-Jun-2026 10:47:29 W/(K*m)  winLength=1 m  winHeight=0.5 m  winThickness=0.007 m  winMaterialDen=2500 kg/m^3  winMaterialCp=787 J/(K*kg)  winAbsorptivity=0.35  winThermalK=1 W/(K*m)  winTransmissivity=0.45  ventLength=0.1 m  ventHeight=0.1 m  extToWallHTC=30 % Parameterized on : 13-Jun-2026 10:47:29 W/(K*m^2)  intToRoomHTC=30 % Parameterized on : 13-Jun-2026 10:47:29 W/(K*m^2)  iniT=300 % Parameterized on : 13-Jun-2026 10:47:29 K
  Floor_A3R5(FireExit_C)Blk : WallSelector_lib/Wall Selector  optWall=wallModelOption.wallOnly  wallLength=1.8288 % Parameterized on : 13-Jun-2026 10:47:15 m  wallHeight=2.1336 % Parameterized on : 13-Jun-2026 10:47:15 m  wallThickness=0.03 % Parameterized on : 13-Jun-2026 10:47:15 m  wallMaterialDen=1400 % Parameterized on : 13-Jun-2026 10:47:29 kg/m^3  wallMaterialCp=1000 % Parameterized on : 13-Jun-2026 10:47:29 J/(K*kg)  wallAbsorptivity=0.5  wallThermalK=0.7 % Parameterized on : 13-Jun-2026 10:47:29 W/(K*m)  winLength=1 m  winHeight=0.5 m  winThickness=0.007 m  winMaterialDen=2500 kg/m^3  winMaterialCp=787 J/(K*kg)  winAbsorptivity=0.35  winThermalK=1 W/(K*m)  winTransmissivity=0.45  ventLength=0.1 m  ventHeight=0.1 m  extToWallHTC=30 % Parameterized on : 13-Jun-2026 10:47:29 W/(K*m^2)  intToRoomHTC=30 % Parameterized on : 13-Jun-2026 10:47:29 W/(K*m^2)  iniT=300 % Parameterized on : 13-Jun-2026 10:47:29 K
  Floor_A3R6(Lobby1_C)Blk : WallSelector_lib/Wall Selector  optWall=wallModelOption.wallOnly  wallLength=2.4384 % Parameterized on : 13-Jun-2026 10:47:15 m  wallHeight=2.4384 % Parameterized on : 13-Jun-2026 10:47:15 m  wallThickness=0.03 % Parameterized on : 13-Jun-2026 10:47:15 m  wallMaterialDen=1400 % Parameterized on : 13-Jun-2026 10:47:29 kg/m^3  wallMaterialCp=1000 % Parameterized on : 13-Jun-2026 10:47:29 J/(K*kg)  wallAbsorptivity=0.5  wallThermalK=0.7 % Parameterized on : 13-Jun-2026 10:47:29 W/(K*m)  winLength=1 m  winHeight=0.5 m  winThickness=0.007 m  winMaterialDen=2500 kg/m^3  winMaterialCp=787 J/(K*kg)  winAbsorptivity=0.35  winThermalK=1 W/(K*m)  winTransmissivity=0.45  ventLength=0.1 m  ventHeight=0.1 m  extToWallHTC=30 % Parameterized on : 13-Jun-2026 10:47:29 W/(K*m^2)  intToRoomHTC=30 % Parameterized on : 13-Jun-2026 10:47:29 W/(K*m^2)  iniT=300 % Parameterized on : 13-Jun-2026 10:47:29 K
  Floor_A3R7(Lobby2_C)Blk : WallSelector_lib/Wall Selector  optWall=wallModelOption.wallOnly  wallLength=2.4384 % Parameterized on : 13-Jun-2026 10:47:15 m  wallHeight=1.524 % Parameterized on : 13-Jun-2026 10:47:15 m  wallThickness=0.03 % Parameterized on : 13-Jun-2026 10:47:15 m  wallMaterialDen=1400 % Parameterized on : 13-Jun-2026 10:47:29 kg/m^3  wallMaterialCp=1000 % Parameterized on : 13-Jun-2026 10:47:29 J/(K*kg)  wallAbsorptivity=0.5  wallThermalK=0.7 % Parameterized on : 13-Jun-2026 10:47:29 W/(K*m)  winLength=1 m  winHeight=0.5 m  winThickness=0.007 m  winMaterialDen=2500 kg/m^3  winMaterialCp=787 J/(K*kg)  winAbsorptivity=0.35  winThermalK=1 W/(K*m)  winTransmissivity=0.45  ventLength=0.1 m  ventHeight=0.1 m  extToWallHTC=30 % Parameterized on : 13-Jun-2026 10:47:29 W/(K*m^2)  intToRoomHTC=30 % Parameterized on : 13-Jun-2026 10:47:29 W/(K*m^2)  iniT=300 % Parameterized on : 13-Jun-2026 10:47:29 K
  Floor_A4R1(LivingRoom_D)Blk : WallSelector_lib/Wall Selector  optWall=wallModelOption.wallOnly  wallLength=2.4384 % Parameterized on : 13-Jun-2026 10:47:15 m  wallHeight=4.572 % Parameterized on : 13-Jun-2026 10:47:15 m  wallThickness=0.03 % Parameterized on : 13-Jun-2026 10:47:15 m  wallMaterialDen=1400 % Parameterized on : 13-Jun-2026 10:47:29 kg/m^3  wallMaterialCp=1000 % Parameterized on : 13-Jun-2026 10:47:29 J/(K*kg)  wallAbsorptivity=0.5  wallThermalK=0.7 % Parameterized on : 13-Jun-2026 10:47:29 W/(K*m)  winLength=1 m  winHeight=0.5 m  winThickness=0.007 m  winMaterialDen=2500 kg/m^3  winMaterialCp=787 J/(K*kg)  winAbsorptivity=0.35  winThermalK=1 W/(K*m)  winTransmissivity=0.45  ventLength=0.1 m  ventHeight=0.1 m  extToWallHTC=30 % Parameterized on : 13-Jun-2026 10:47:29 W/(K*m^2)  intToRoomHTC=30 % Parameterized on : 13-Jun-2026 10:47:29 W/(K*m^2)  iniT=300 % Parameterized on : 13-Jun-2026 10:47:29 K
  Floor_A4R2(Bedroom_D)Blk : WallSelector_lib/Wall Selector  optWall=wallModelOption.wallOnly  wallLength=4.2672 % Parameterized on : 13-Jun-2026 10:47:15 m  wallHeight=4.572 % Parameterized on : 13-Jun-2026 10:47:15 m  wallThickness=0.03 % Parameterized on : 13-Jun-2026 10:47:15 m  wallMaterialDen=1400 % Parameterized on : 13-Jun-2026 10:47:29 kg/m^3  wallMaterialCp=1000 % Parameterized on : 13-Jun-2026 10:47:29 J/(K*kg)  wallAbsorptivity=0.5  wallThermalK=0.7 % Parameterized on : 13-Jun-2026 10:47:29 W/(K*m)  winLength=1 m  winHeight=0.5 m  winThickness=0.007 m  winMaterialDen=2500 kg/m^3  winMaterialCp=787 J/(K*kg)  winAbsorptivity=0.35  winThermalK=1 W/(K*m)  winTransmissivity=0.45  ventLength=0.1 m  ventHeight=0.1 m  extToWallHTC=30 % Parameterized on : 13-Jun-2026 10:47:29 W/(K*m^2)  intToRoomHTC=30 % Parameterized on : 13-Jun-2026 10:47:29 W/(K*m^2)  iniT=300 % Parameterized on : 13-Jun-2026 10:47:29 K
  Floor_A4R3(Kitchen_D)Blk : WallSelector_lib/Wall Selector  optWall=wallModelOption.wallOnly  wallLength=2.7432 % Parameterized on : 13-Jun-2026 10:47:15 m  wallHeight=3.9624 % Parameterized on : 13-Jun-2026 10:47:15 m  wallThickness=0.03 % Parameterized on : 13-Jun-2026 10:47:15 m  wallMaterialDen=1400 % Parameterized on : 13-Jun-2026 10:47:29 kg/m^3  wallMaterialCp=1000 % Parameterized on : 13-Jun-2026 10:47:29 J/(K*kg)  wallAbsorptivity=0.5  wallThermalK=0.7 % Parameterized on : 13-Jun-2026 10:47:29 W/(K*m)  winLength=1 m  winHeight=0.5 m  winThickness=0.007 m  winMaterialDen=2500 kg/m^3  winMaterialCp=787 J/(K*kg)  winAbsorptivity=0.35  winThermalK=1 W/(K*m)  winTransmissivity=0.45  ventLength=0.1 m  ventHeight=0.1 m  extToWallHTC=30 % Parameterized on : 13-Jun-2026 10:47:29 W/(K*m^2)  intToRoomHTC=30 % Parameterized on : 13-Jun-2026 10:47:29 W/(K*m^2)  iniT=300 % Parameterized on : 13-Jun-2026 10:47:29 K
  Floor_A4R4(Bathroom_D)Blk : WallSelector_lib/Wall Selector  optWall=wallModelOption.wallOnly  wallLength=2.4384 % Parameterized on : 13-Jun-2026 10:47:15 m  wallHeight=3.6576 % Parameterized on : 13-Jun-2026 10:47:15 m  wallThickness=0.03 % Parameterized on : 13-Jun-2026 10:47:15 m  wallMaterialDen=1400 % Parameterized on : 13-Jun-2026 10:47:29 kg/m^3  wallMaterialCp=1000 % Parameterized on : 13-Jun-2026 10:47:29 J/(K*kg)  wallAbsorptivity=0.5  wallThermalK=0.7 % Parameterized on : 13-Jun-2026 10:47:29 W/(K*m)  winLength=1 m  winHeight=0.5 m  winThickness=0.007 m  winMaterialDen=2500 kg/m^3  winMaterialCp=787 J/(K*kg)  winAbsorptivity=0.35  winThermalK=1 W/(K*m)  winTransmissivity=0.45  ventLength=0.1 m  ventHeight=0.1 m  extToWallHTC=30 % Parameterized on : 13-Jun-2026 10:47:29 W/(K*m^2)  intToRoomHTC=30 % Parameterized on : 13-Jun-2026 10:47:29 W/(K*m^2)  iniT=300 % Parameterized on : 13-Jun-2026 10:47:29 K
  Floor_A4R5(FireExit_D)Blk : WallSelector_lib/Wall Selector  optWall=wallModelOption.wallOnly  wallLength=1.8288 % Parameterized on : 13-Jun-2026 10:47:15 m  wallHeight=2.1336 % Parameterized on : 13-Jun-2026 10:47:15 m  wallThickness=0.03 % Parameterized on : 13-Jun-2026 10:47:15 m  wallMaterialDen=1400 % Parameterized on : 13-Jun-2026 10:47:29 kg/m^3  wallMaterialCp=1000 % Parameterized on : 13-Jun-2026 10:47:29 J/(K*kg)  wallAbsorptivity=0.5  wallThermalK=0.7 % Parameterized on : 13-Jun-2026 10:47:29 W/(K*m)  winLength=1 m  winHeight=0.5 m  winThickness=0.007 m  winMaterialDen=2500 kg/m^3  winMaterialCp=787 J/(K*kg)  winAbsorptivity=0.35  winThermalK=1 W/(K*m)  winTransmissivity=0.45  ventLength=0.1 m  ventHeight=0.1 m  extToWallHTC=30 % Parameterized on : 13-Jun-2026 10:47:29 W/(K*m^2)  intToRoomHTC=30 % Parameterized on : 13-Jun-2026 10:47:29 W/(K*m^2)  iniT=300 % Parameterized on : 13-Jun-2026 10:47:29 K
  Floor_A4R6(Lobby1_D)Blk : WallSelector_lib/Wall Selector  optWall=wallModelOption.wallOnly  wallLength=2.4384 % Parameterized on : 13-Jun-2026 10:47:15 m  wallHeight=2.4384 % Parameterized on : 13-Jun-2026 10:47:15 m  wallThickness=0.03 % Parameterized on : 13-Jun-2026 10:47:15 m  wallMaterialDen=1400 % Parameterized on : 13-Jun-2026 10:47:29 kg/m^3  wallMaterialCp=1000 % Parameterized on : 13-Jun-2026 10:47:29 J/(K*kg)  wallAbsorptivity=0.5  wallThermalK=0.7 % Parameterized on : 13-Jun-2026 10:47:29 W/(K*m)  winLength=1 m  winHeight=0.5 m  winThickness=0.007 m  winMaterialDen=2500 kg/m^3  winMaterialCp=787 J/(K*kg)  winAbsorptivity=0.35  winThermalK=1 W/(K*m)  winTransmissivity=0.45  ventLength=0.1 m  ventHeight=0.1 m  extToWallHTC=30 % Parameterized on : 13-Jun-2026 10:47:29 W/(K*m^2)  intToRoomHTC=30 % Parameterized on : 13-Jun-2026 10:47:29 W/(K*m^2)  iniT=300 % Parameterized on : 13-Jun-2026 10:47:29 K
  Floor_A4R7(Lobby2_D)Blk : WallSelector_lib/Wall Selector  optWall=wallModelOption.wallOnly  wallLength=2.4384 % Parameterized on : 13-Jun-2026 10:47:15 m  wallHeight=1.524 % Parameterized on : 13-Jun-2026 10:47:15 m  wallThickness=0.03 % Parameterized on : 13-Jun-2026 10:47:15 m  wallMaterialDen=1400 % Parameterized on : 13-Jun-2026 10:47:29 kg/m^3  wallMaterialCp=1000 % Parameterized on : 13-Jun-2026 10:47:29 J/(K*kg)  wallAbsorptivity=0.5  wallThermalK=0.7 % Parameterized on : 13-Jun-2026 10:47:29 W/(K*m)  winLength=1 m  winHeight=0.5 m  winThickness=0.007 m  winMaterialDen=2500 kg/m^3  winMaterialCp=787 J/(K*kg)  winAbsorptivity=0.35  winThermalK=1 W/(K*m)  winTransmissivity=0.45  ventLength=0.1 m  ventHeight=0.1 m  extToWallHTC=30 % Parameterized on : 13-Jun-2026 10:47:29 W/(K*m^2)  intToRoomHTC=30 % Parameterized on : 13-Jun-2026 10:47:29 W/(K*m^2)  iniT=300 % Parameterized on : 13-Jun-2026 10:47:29 K
  Top : PMIOPort  Side=Left
  Bottom : PMIOPort  Port=2  Side=Right
  connections:
  ArrayTop/RConn1 -- Top/RConn1
  Floor_A1R1(LivingRoom_A)Blk/LConn1 -- ArrayTop/LConn1
  Floor_A1R2(Bedroom_A)Blk/LConn1 -- ArrayTop/LConn2
  Floor_A1R3(Kitchen_A)Blk/LConn1 -- ArrayTop/LConn3
  Floor_A1R4(Bathroom_A)Blk/LConn1 -- ArrayTop/LConn4
  Floor_A1R5(FireExit_A)Blk/LConn1 -- ArrayTop/LConn5
  Floor_A1R6(Lobby1_A)Blk/LConn1 -- ArrayTop/LConn6
  Floor_A1R7(Lobby2_A)Blk/LConn1 -- ArrayTop/LConn7
  Floor_A2R1(LivingRoom_B)Blk/LConn1 -- ArrayTop/LConn8
  Floor_A2R2(Bedroom_B)Blk/LConn1 -- ArrayTop/LConn9
  Floor_A2R3(Kitchen_B)Blk/LConn1 -- ArrayTop/LConn10
  Floor_A2R4(Bathroom_B)Blk/LConn1 -- ArrayTop/LConn11
  Floor_A2R5(FireExit_B)Blk/LConn1 -- ArrayTop/LConn12
  Floor_A2R6(Lobby1_B)Blk/LConn1 -- ArrayTop/LConn13
  Floor_A2R7(Lobby2_B)Blk/LConn1 -- ArrayTop/LConn14
  Floor_A3R1(LivingRoom_C)Blk/LConn1 -- ArrayTop/LConn15
  Floor_A3R2(Bedroom_C)Blk/LConn1 -- ArrayTop/LConn16
  Floor_A3R3(Kitchen_C)Blk/LConn1 -- ArrayTop/LConn17
  Floor_A3R4(Bathroom_C)Blk/LConn1 -- ArrayTop/LConn18
  Floor_A3R5(FireExit_C)Blk/LConn1 -- ArrayTop/LConn19
  Floor_A3R6(Lobby1_C)Blk/LConn1 -- ArrayTop/LConn20
  Floor_A3R7(Lobby2_C)Blk/LConn1 -- ArrayTop/LConn21
  Floor_A4R1(LivingRoom_D)Blk/LConn1 -- ArrayTop/LConn22
  Floor_A4R2(Bedroom_D)Blk/LConn1 -- ArrayTop/LConn23
  Floor_A4R3(Kitchen_D)Blk/LConn1 -- ArrayTop/LConn24
  Floor_A4R4(Bathroom_D)Blk/LConn1 -- ArrayTop/LConn25
  Floor_A4R5(FireExit_D)Blk/LConn1 -- ArrayTop/LConn26
  Floor_A4R6(Lobby1_D)Blk/LConn1 -- ArrayTop/LConn27
  Floor_A4R7(Lobby2_D)Blk/LConn1 -- ArrayTop/LConn28
  ArrayBottom/RConn1 -- Bottom/RConn1
  Floor_A1R1(LivingRoom_A)Blk/RConn1 -- ArrayBottom/LConn1
  Floor_A1R2(Bedroom_A)Blk/RConn1 -- ArrayBottom/LConn2
  Floor_A1R3(Kitchen_A)Blk/RConn1 -- ArrayBottom/LConn3
  Floor_A1R4(Bathroom_A)Blk/RConn1 -- ArrayBottom/LConn4
  Floor_A1R5(FireExit_A)Blk/RConn1 -- ArrayBottom/LConn5
  Floor_A1R6(Lobby1_A)Blk/RConn1 -- ArrayBottom/LConn6
  Floor_A1R7(Lobby2_A)Blk/RConn1 -- ArrayBottom/LConn7
  Floor_A2R1(LivingRoom_B)Blk/RConn1 -- ArrayBottom/LConn8
  Floor_A2R2(Bedroom_B)Blk/RConn1 -- ArrayBottom/LConn9
  Floor_A2R3(Kitchen_B)Blk/RConn1 -- ArrayBottom/LConn10
  Floor_A2R4(Bathroom_B)Blk/RConn1 -- ArrayBottom/LConn11
  Floor_A2R5(FireExit_B)Blk/RConn1 -- ArrayBottom/LConn12
  Floor_A2R6(Lobby1_B)Blk/RConn1 -- ArrayBottom/LConn13
  Floor_A2R7(Lobby2_B)Blk/RConn1 -- ArrayBottom/LConn14
  Floor_A3R1(LivingRoom_C)Blk/RConn1 -- ArrayBottom/LConn15
  Floor_A3R2(Bedroom_C)Blk/RConn1 -- ArrayBottom/LConn16
  Floor_A3R3(Kitchen_C)Blk/RConn1 -- ArrayBottom/LConn17
  Floor_A3R4(Bathroom_C)Blk/RConn1 -- ArrayBottom/LConn18
  Floor_A3R5(FireExit_C)Blk/RConn1 -- ArrayBottom/LConn19
  Floor_A3R6(Lobby1_C)Blk/RConn1 -- ArrayBottom/LConn20
  Floor_A3R7(Lobby2_C)Blk/RConn1 -- ArrayBottom/LConn21
  Floor_A4R1(LivingRoom_D)Blk/RConn1 -- ArrayBottom/LConn22
  Floor_A4R2(Bedroom_D)Blk/RConn1 -- ArrayBottom/LConn23
  Floor_A4R3(Kitchen_D)Blk/RConn1 -- ArrayBottom/LConn24
  Floor_A4R4(Bathroom_D)Blk/RConn1 -- ArrayBottom/LConn25
  Floor_A4R5(FireExit_D)Blk/RConn1 -- ArrayBottom/LConn26
  Floor_A4R6(Lobby1_D)Blk/RConn1 -- ArrayBottom/LConn27
  Floor_A4R7(Lobby2_D)Blk/RConn1 -- ArrayBottom/LConn28
